simulink model "untitled1"  (R2024b)
settings: Solver=FixedStepAuto  StartTime=0.0  StopTime=15.0  FixedStep=0.01  RelTol=1e-3
libraries: fuzblock x2
settings Model: Creator=l18  LastModifiedBy=l18

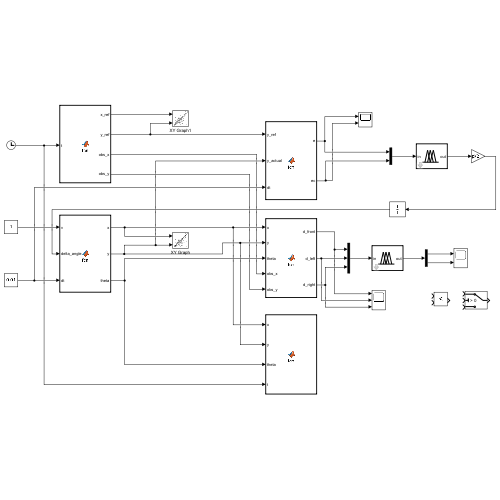
[thumbnail: Simulink's stored preview of the top-level diagram]
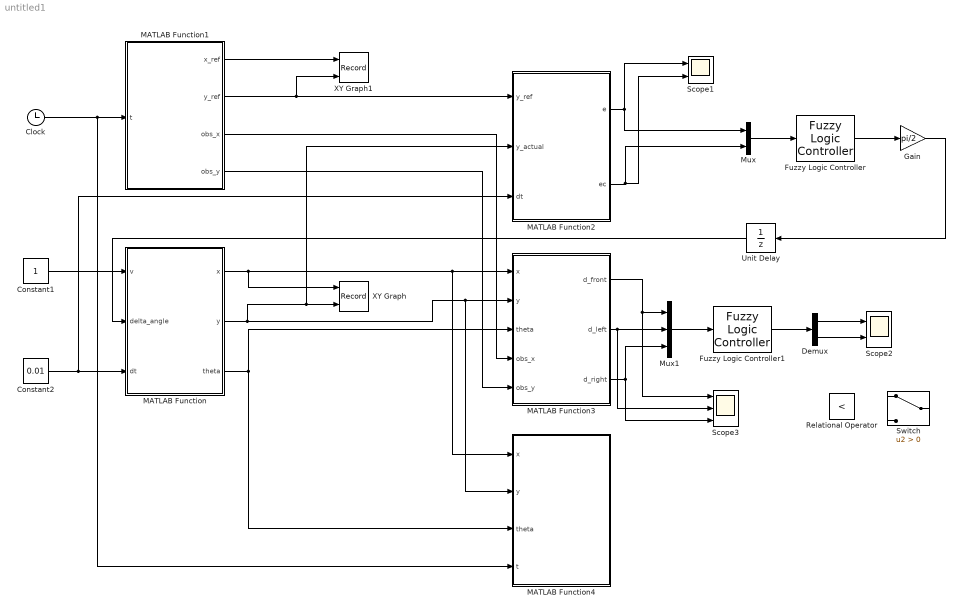
== system untitled1 ==
  Clock : Clock
  Constant1 : Constant
  Constant2 : Constant  Value=0.01
  Demux : Demux  Outputs=2
  Fuzzy Logic Controller : fuzblock/Fuzzy Logic  Controller  Description=循迹模糊控制器  FIS='tracking_fis.fis'  OutputSampleNumber=101  DataType=double  FuzzifiedInputs=off  RuleFiringStrengths=off  RuleOutputs=off  AggregatedOutputs=off  SimulateUsing=Interpreted execution  OutOfRangeInputValueMessage=warning  NoRuleFiredMessage=warning  EmptyOutputFuzzySetMessage=warning
  Fuzzy Logic Controller1 : fuzblock/Fuzzy Logic  Controller  Description=避障模糊控制器  FIS='avoidance_v2.fis'  OutputSampleNumber=101  DataType=double  FuzzifiedInputs=off  RuleFiringStrengths=off  RuleOutputs=off  AggregatedOutputs=off  SimulateUsing=Interpreted execution  OutOfRangeInputValueMessage=warning  NoRuleFiredMessage=warning  EmptyOutputFuzzySetMessage=warning
  Gain : Gain  Gain=pi/2
  MATLAB Function : MATLAB Function  TreatAsAtomicUnit=on
  MATLAB Function1 : MATLAB Function  TreatAsAtomicUnit=on
  MATLAB Function2 : MATLAB Function  TreatAsAtomicUnit=on
  MATLAB Function3 : MATLAB Function  TreatAsAtomicUnit=on
  MATLAB Function4 : MATLAB Function  TreatAsAtomicUnit=on
  Mux : Mux  Inputs=2
  Mux1 : Mux  Inputs=3
  Relational Operator : RelationalOperator  Operator=<  OutDataTypeStr=boolean  RndMeth=Simplest  InputSameDT=off
  Scope1 : Scope  NumInputPorts=2
  Scope2 : Scope  NumInputPorts=2
  Scope3 : Scope  NumInputPorts=3
  Switch : Switch  Criteria=u2 > Threshold  SaturateOnIntegerOverflow=off  InputSameDT=off
  Unit Delay : UnitDelay  SampleTime=-1  HasFrameUpgradeWarning=on
  XY Graph : Record  FileSettingsInternal="{\"entries\":[{\"content\":{\"excelSettings\":{\"content\":{},\"type\":\"Streamout.ExcelSettings\"}},\"type\":\"Streamout.FileSettingStorage\",\"uuid\":\"\"}],\"packageUris\":[\"http:\\/\\/schema.mathworks.com\\/mf0\\/streamout_blocks\\/R2020a\"],\"version\":\"1.0\"}"  Layout=[1 1]  SignalsInternal="{\"entries\":[{\"content\":{},\"type\":\"RecordBlkView.InputSignals\",\"uuid\":\"\"}],\"packageUris\":[\"http:\\/\\/schema.mathworks.com\\/mf0\\/streamout_blocks\\/R2020a\"],\"version\":\"1.0\"}"  VisualizationBindings="{\"xyplotplugin\":{\"info\":[{\"series\":[{\"bindingParametersList\":[{\"parameter\":\"X-Axis\",\"signalID\":52,\"signalName\":\"MATLAB Function:1\"},{\"parameter\":\"Y-Axis\",\"signalID\":56,\"signalName\":\"MATLAB Function:2\"}],\"seriesID\":0}],\"subplotID\":1}]}}"  CompatibilityTag=XY
  XY Graph1 : Record  FileSettingsInternal="{\"entries\":[{\"content\":{\"excelSettings\":{\"content\":{},\"type\":\"Streamout.ExcelSettings\"}},\"type\":\"Streamout.FileSettingStorage\",\"uuid\":\"\"}],\"packageUris\":[\"http:\\/\\/schema.mathworks.com\\/mf0\\/streamout_blocks\\/R2020a\"],\"version\":\"1.0\"}"  Layout=[1 1]  SignalsInternal="{\"entries\":[{\"content\":{},\"type\":\"RecordBlkView.InputSignals\",\"uuid\":\"\"}],\"packageUris\":[\"http:\\/\\/schema.mathworks.com\\/mf0\\/streamout_blocks\\/R2020a\"],\"version\":\"1.0\"}"  VisualizationBindings="{\"xyplotplugin\":{\"info\":[{\"series\":[{\"bindingParametersList\":[{\"parameter\":\"X-Axis\",\"signalID\":60,\"signalName\":\"MATLAB Function1:1\"},{\"parameter\":\"Y-Axis\",\"signalID\":64,\"signalName\":\"MATLAB Function1:2\"}],\"seriesID\":0}],\"subplotID\":1}]}}"  CompatibilityTag=XY
  wires:
  Constant2/1 -> MATLAB Function2/3(dt), MATLAB Function/3(dt)
  Constant1/1 -> MATLAB Function/1(v)
  MATLAB Function/1(x) -> MATLAB Function4/1(x), MATLAB Function3/1(x), XY Graph/1
  MATLAB Function/2(y) -> MATLAB Function4/2(y), MATLAB Function3/2(y), XY Graph/2, MATLAB Function2/2(y_actual)
  MATLAB Function/3(theta) -> MATLAB Function4/3(theta), MATLAB Function3/3(theta)
  Clock/1 -> MATLAB Function4/4(t), MATLAB Function1/1(t)
  MATLAB Function1/2(y_ref) -> XY Graph1/2, MATLAB Function2/1(y_ref)
  MATLAB Function1/3(obs_x) -> MATLAB Function3/4(obs_x)
  MATLAB Function1/4(obs_y) -> MATLAB Function3/5(obs_y)
  MATLAB Function2/1(e) -> Scope1/1, Mux/1
  MATLAB Function2/2(ec) -> Scope1/2, Mux/2
  Mux/1 -> Fuzzy Logic Controller/1
  MATLAB Function3/1(d_front) -> Scope3/1, Mux1/1
  MATLAB Function3/2(d_left) -> Scope3/2, Mux1/2
  MATLAB Function3/3(d_right) -> Scope3/3, Mux1/3
  Mux1/1 -> Fuzzy Logic Controller1/1
  MATLAB Function1/1(x_ref) -> XY Graph1/1
  Fuzzy Logic Controller/1 -> Gain/1
  Gain/1 -> Unit Delay/1
  Unit Delay/1 -> MATLAB Function/2(delta_angle)
  Fuzzy Logic Controller1/1 -> Demux/1
  Demux/2 -> Scope2/2
  Demux/1 -> Scope2/1

== matlab function untitled1/MATLAB Function1 ==
  settings: description=生成循迹路线
  data: x_ref output; t input; y_ref output; obs_x output; obs_y output
function [x_ref, y_ref, obs_x, obs_y] = fcn(t)
    v_ref = 1.0;
    x_ref = v_ref * t;
    if t < 5
        y_ref = 0; % 前5秒直线
    else
        y_ref = 1 * sin(1* (x_ref - 5)); % 5秒后S弯
    end
    
    % 设置障碍物：如果在特定时间后，让障碍物横向移动（动态障碍）
    obs_x = 8; 
    obs_y = 0.5;
    % if t > 6
    %     obs_y = 0.5 + 0.2 * sin(2*t); % 6秒后变成动态障碍物
    % else
    %     obs_y = 0.5; % 静态障碍物
    % end
end

== matlab function untitled1/MATLAB Function ==
  settings: sampleTime=0.01  description=小车运动模型
  data: x output; v input; y output; delta_angle input; dt input; theta output
function [x, y, theta] = fcn(v, delta_angle, dt)
    persistent x_s y_s;
    if isempty(x_s)
        x_s = 0; y_s = 0;
    end
    
    % 把 delta_angle 当成直接的角度指令，不再积分！
    % 假设 v 是线速度，x、y 是坐标
    theta = delta_angle;  % 直接赋值给车头方向
    
    x_s = x_s + v * cos(theta) * dt;
    y_s = y_s + v * sin(theta) * dt;
    
    x = x_s; y = y_s;
end

== matlab function untitled1/MATLAB Function2 ==
  settings: sampleTime=0.01  description=循迹传感器模拟
  data: e output; y_ref input; ec output; y_actual input; dt input



function [e, ec] = fcn(y_ref, y_actual, dt)
    % 1. 计算原始横向偏差 (单位：米)
    e_raw = y_ref - y_actual; 
    
    % 2. 计算原始偏差变化率
    persistent e_prev;
    if isempty(e_prev)
        e_prev = 0; 
    end
    ec_raw = (e_raw - e_prev) / dt;
    e_prev = e_raw;
    
    % ==========================================
    % 3. 核心步骤：归一化 (映射到 [-1, 1] 的模糊论域)
    % 假设你的赛道最大可能偏离为 1.0 米，速度变化极值为 5 m/s
    % 你可以根据自己的场地大小修改这两个分母
    % ==========================================
    e_max = 1.0;  % 误差最大值
    ec_max = 5.0; % 误差变化率最大值
    
    e = e_raw / e_max;
    ec = ec_raw / ec_max;
    
    % 4. 强制限幅：防止小车失控飞出赛道时输入超纲 ([-1, 1])
    if e > 1, e = 1; elseif e < -1, e = -1; end
    if ec > 1, ec = 1; elseif ec < -1, ec = -1; end
end

== matlab function untitled1/MATLAB Function3 ==
  settings: description=避障传感器模拟
  data: d_front output; x input; d_left output; y input; theta input; obs_x input; obs_y input; d_right output
function [d_front, d_left, d_right] = fcn(x, y, theta, obs_x, obs_y)
    % 1. 计算小车到障碍物的绝对距离和相对角度
    dx = obs_x - x;
    dy = obs_y - y;
    dist = sqrt(dx^2 + dy^2);
    
    % 计算障碍物相对于世界坐标系的偏角
    angle_to_obs = atan2(dy, dx);
    
    % 计算障碍物相对于小车车头(theta)的偏角
    rel_angle = angle_to_obs - theta;
    % 归一化到 -pi/2 到 pi/2 之间
    rel_angle = atan2(sin(rel_angle), cos(rel_angle));
    
    % 2. 设定雷达的最大探测范围（单位：米）
    max_range = 1.0;
    
    % 默认三个方向都是安全的（最大距离）
    d_front = max_range;
    d_left = max_range;
    d_right = max_range;
    
    % 3. 划分探测扇区（注意：这里的角度划分可根据你的实际需求微调）
    % 前方：正负 45度以内 (-pi/4 到 pi/4)
    if abs(rel_angle) < pi/4
        d_front = dist;
    % 左侧：45度 到 135度 (pi/4 到 3*pi/4)
    elseif rel_angle >= pi/4 && rel_angle < pi/2
        d_left = dist;
    % 右侧：-45度 到 -135度 (-pi/4 到 -3*pi/4)
    elseif rel_angle <= -pi/4 && rel_angle > pi/2
        d_right = dist;
    end
    
    % 4. 归一化处理（模糊控制器的论域是 0~1）
    % 限制物理距离不超过最大探测范围
    d_front = min(d_front, max_range) / max_range;
    d_left  = min(d_left, max_range) / max_range;
    d_right = min(d_right, max_range) / max_range;
end

== matlab function untitled1/MATLAB Function4 ==
  settings: description=小车轨迹动画显示
  data: x input; y input; theta input; t input
function fcn(x, y, theta, t)
    % 注意：输入增加了 t（仿真时间）
    persistent h_car h_trajectory h_time
    
    % 1. 初始化画布（只在仿真第一步执行）
    if isempty(h_car)
        figure('Name', 'Car Animation', 'NumberTitle', 'off');
        hold on; grid on; axis equal;
        xlabel('X (m)'); ylabel('Y (m)');
        xlim([-2, 15]); ylim([-5, 5]); 
        
        % 画小车
        car_x = [-0.2, 0.2, 0.2, -0.2, -0.2];
        car_y = [-0.1, -0.1, 0.1, 0.1, -0.1];
        h_car = plot(car_x + x, car_y + y, 'r-', 'LineWidth', 2);
        
        % 画轨迹线
        h_trajectory = plot(x, y, 'b-', 'LineWidth', 1);
        
        % 新增：创建一个文本对象显示时间（位置放在左上角 X=-1.8, Y=4.5）
        h_time = text(-1.8, 4.5, 'Time: 0.00 s', 'FontSize', 12, 'FontWeight', 'bold', 'Color', 'k');
    end
    
    % 2. 计算小车当前姿态的坐标
    car_x = [-0.2, 0.2, 0.2, -0.2, -0.2];
    car_y = [-0.1, -0.1, 0.1, 0.1, -0.1];
    R = [cos(theta), -sin(theta); sin(theta), cos(theta)];
    global_coords = R * [car_x; car_y];
    new_x = global_coords(1, :) + x;
    new_y = global_coords(2, :) + y;
    
    % 3. 更新小车位置
    set(h_car, 'XData', new_x, 'YData', new_y);
    
    % 4. 更新轨迹
    set(h_trajectory, 'XData', [get(h_trajectory, 'XData'), x], ...
                      'YData', [get(h_trajectory, 'YData'), y]);
    
    % 5. 新增：更新文本内容
    set(h_time, 'String', sprintf('Time: %.2f s', t));
    
    % 6. 强制屏幕刷新
    drawnow; 
end
